simulink model "surrogate_model_9"  (R2026a)
settings: Solver=VariableStepAuto
settings Model: Creator=shuki  LastModifiedBy=shuki

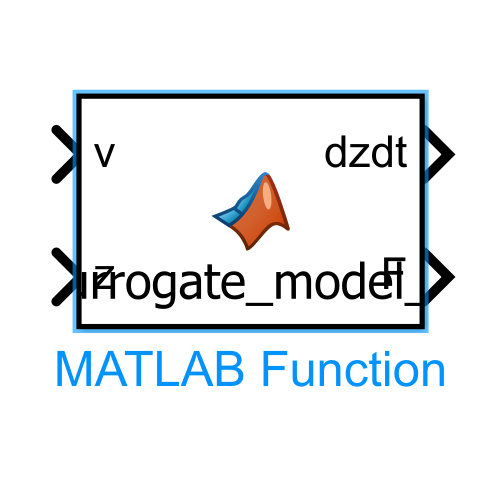
[thumbnail: Simulink's stored preview of the top-level diagram]
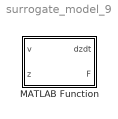
== system surrogate_model_9 ==
  MATLAB Function : MATLAB Function  TreatAsAtomicUnit=on

== matlab function surrogate_model_9/MATLAB Function ==
  data: dzdt output; F output; v input; z input
function [dzdt, F] = surrogate_model_9(v, z)

    S0 = 10^5;
    C1 = 3.32089;
    C2 = 0.47075325;
    C3 = 2.4649878;

    dzdt = v - z*( (abs(S0*v + C1) + abs(C1 - S0*v) )*C2 - C3);

    F = 10^5 * z + 316.2277 * dzdt + 0.4 * v;

end
